simulink model "ASM_Traffic"  (R2026a)
settings: Solver=ode1  StartTime=SIM.tstart.v  StopTime=SIM.tend.v  FixedStep=SIM.StepSize.v
PostLoadFcn:
  | if any(exist('dsrtsu_mdlpostloadfcn', 'file') ~= 0), dsrtsu_mdlpostloadfcn('Execute', bdroot); end
  | try, asm_mdl_postloadfcn(bdroot, 'UpdateModel', 3600); catch, disp(lasterr); end,
InitFcn:
  | , if any(exist('rtifpga_mdlclblib', 'file') ~= 0), rtifpga_mdlclblib('Init', bdroot); end,
  | , if any(exist('dsmpb_private', 'file') ~= 0), dsmpb_private('dsmpb_mdlclblib', 'Init', bdroot); end,
model workspace (MAT data in the model file):
  asmReferencePath = [0 0.01 0.02 0.03 0.04 0.05 0.06 0.07 0.08 0.09 0.1 0.11 ... (350007 elements, 50001x7)]
  roadBounds : Simulink.Parameter (value not decoded)
  safetyAxes : Simulink.Parameter (value not decoded)
undefined symbols (not defined in the file): _to_, a0b2, ASM_BrakeHydraulics_DemoSystems, ASM_VehicleDynamics_DemoSystems, b98103fe8ad365046cd0, BrakeCircuit, controllerConfig, CPT, Crankshaft, DiscIntNeverNeededParam, dsmsi, FinalDriveAssembly, MDL, ModeSignals, mu, Pos_BrakePedal_Maneuver, rad, RefSignals, roadFamilyData, roadFamilyId, s_to_rpm, SIM, SoftECU, Suspension, Tire, Transmission
libraries: ASM_Traffic_lib x135, simulink x98, ASM_Utils_lib x77, ASM_VehicleDynamics_lib x70, ASM_Environment_lib x22, dsmpblib x20, dsmsilib x15, MDLD_Utils_lib x10, ASM_BrakeHydraulics_lib x3, sl_discontinuities x2
(part 40 of 65)

== system ASM_Traffic/Environment/Road/UserInterface/PAR_Plant/Pos_CP_CoorsSys_E[:][x;y][m] ==
  Pos_CP[x;y][m] : Inport
  Active_CP_VehDyn_Trailer[] : Inport  Port=2
  Bus Selector : BusSelector  OutputSignals=Pos_CP_FL_CoorSys_E[x;y][m],Pos_CP_FR_CoorSys_E[x;y][m],Pos_CP_RL_CoorSys_E[x;y][m],Pos_CP_RL2_CoorSys_E[x;y][m],Pos_CP_RR_CoorSys_E[x;y][m],Pos_CP_RR2_CoorSys_E[x;y][m],Pos_CP_R2L_CoorSys_E[x;y][m],Pos_CP_R2L2_CoorSys_E[x;y][m],Pos_CP_R2R_CoorSys_E[x;y][m],Pos_CP_R2R2_CoorSys_E[x;y][m],Pos_CP_FL_Trailer_CoorSys_E[x;y][m],Pos_CP_FL2_Trailer_CoorSys_E[x;y][m],Pos_CP_FR_Trailer_CoorSys_E[x;y][m],Pos_CP_FR2_Trailer_CoorSys_E[x;y][m],Pos_CP_RL_Trailer_CoorSys_E[x;y][m],Pos_CP_RL2_Trailer_CoorSys_E[x;y][m],Pos_CP_RR_Trailer_CoorSys_E[x;y][m],Pos_CP_RR2_Trailer_CoorSys_E[x;y][m],Pos_CP_R2L_Trailer_CoorSys_E[x;y][m],Pos_CP_R2L2_Trailer_CoorSys_E[x;y][m],Pos_CP_R2R_Trailer_CoorSys_E[x;y][m],Pos_CP_R2R2_Trailer_CoorSys_E[x;y][m],Pos_CP_Front_CoorSys_E[x;y][m],Pos_CP_Rear_CoorSys_E[x;y][m]
  Mux : Mux  Inputs=24
  Selector : Selector  IndexOptions=Index vector (port)  Indices=[1 3]  OutputSizes=1
  Pos_CP_CoorsSys_E[:][x;y][m] : Outport  VectorParamsAs1DForOutWhenUnconnected=off
  wires:
  Bus Selector/24 -> Mux/24  "<Pos_CP_Rear_CoorSys_E[x;y][m]>"
  Bus Selector/23 -> Mux/23  "<Pos_CP_Front_CoorSys_E[x;y][m]>"
  Selector/1 -> Pos_CP_CoorsSys_E[:][x;y][m]/1
  Active_CP_VehDyn_Trailer[]/1 -> Selector/2
  Pos_CP[x;y][m]/1 -> Bus Selector/1
  Bus Selector/1 -> Mux/1  "<Pos_CP_FL_CoorSys_E[x;y][m]>"
  Bus Selector/2 -> Mux/2  "<Pos_CP_FR_CoorSys_E[x;y][m]>"
  Bus Selector/3 -> Mux/3  "<Pos_CP_RL_CoorSys_E[x;y][m]>"
  Bus Selector/4 -> Mux/4  "<Pos_CP_RL2_CoorSys_E[x;y][m]>"
  Bus Selector/5 -> Mux/5  "<Pos_CP_RR_CoorSys_E[x;y][m]>"
  Bus Selector/6 -> Mux/6  "<Pos_CP_RR2_CoorSys_E[x;y][m]>"
  Bus Selector/7 -> Mux/7  "<Pos_CP_R2L_CoorSys_E[x;y][m]>"
  Bus Selector/8 -> Mux/8  "<Pos_CP_R2L2_CoorSys_E[x;y][m]>"
  Bus Selector/9 -> Mux/9  "<Pos_CP_R2R_CoorSys_E[x;y][m]>"
  Bus Selector/10 -> Mux/10  "<Pos_CP_R2R2_CoorSys_E[x;y][m]>"
  Bus Selector/11 -> Mux/11  "<Pos_CP_FL_Trailer_CoorSys_E[x;y][m]>"
  Bus Selector/12 -> Mux/12  "<Pos_CP_FL2_Trailer_CoorSys_E[x;y][m]>"
  Bus Selector/13 -> Mux/13  "<Pos_CP_FR_Trailer_CoorSys_E[x;y][m]>"
  Bus Selector/14 -> Mux/14  "<Pos_CP_FR2_Trailer_CoorSys_E[x;y][m]>"
  Bus Selector/15 -> Mux/15  "<Pos_CP_RL_Trailer_CoorSys_E[x;y][m]>"
  Bus Selector/16 -> Mux/16  "<Pos_CP_RL2_Trailer_CoorSys_E[x;y][m]>"
  Bus Selector/17 -> Mux/17  "<Pos_CP_RR_Trailer_CoorSys_E[x;y][m]>"
  Bus Selector/18 -> Mux/18  "<Pos_CP_RR2_Trailer_CoorSys_E[x;y][m]>"
  Bus Selector/19 -> Mux/19  "<Pos_CP_R2L_Trailer_CoorSys_E[x;y][m]>"
  Bus Selector/20 -> Mux/20  "<Pos_CP_R2L2_Trailer_CoorSys_E[x;y][m]>"
  Bus Selector/21 -> Mux/21  "<Pos_CP_R2R_Trailer_CoorSys_E[x;y][m]>"
  Bus Selector/22 -> Mux/22  "<Pos_CP_R2R2_Trailer_CoorSys_E[x;y][m]>"
  Mux/1 -> Selector/1

== system ASM_Traffic/Environment/Sensors/PlantModel/Collision_Sensor/ASMSignalCollector ==
  Bus Creator3 : BusCreator  Inputs=1
  tag scope: ASMBUS_Environment_Traffic_Sensors_Collision_Sensor=scoped
  wires:
  [ASMBUS_Traf_Sensors_Collision_Sensor_1] -> Bus Creator3/1  "Collision_Sensor_1"
  Bus Creator3/1 -> [ASMBUS_Environment_Traffic_Sensors_Collision_Sensor]  "Collision_Sensor"

== system ASM_Traffic/Environment/Sensors/PlantModel/Collision_Sensor/Enable_Collision_Sensor ==
  Enable_In[0Off|1On] : Inport
  Constant : Constant  Value=0.5  SampleTime=-1
  Constant1 : Constant  SampleTime=-1
  Constant2 : Constant  Value=0  SampleTime=-1
  Enable_Sensor : Gain
  Multiport Switch : MultiPortSwitch  DataPortOrder=Zero-based contiguous  Inputs=2  zeroidx=on  SaturateOnIntegerOverflow=off  InputSameDT=off
  Relational Operator : RelationalOperator  Operator=>  OutDataTypeStr=boolean  InputSameDT=off
  Enable_Out[0Off|1On] : Outport  VectorParamsAs1DForOutWhenUnconnected=off
  wires:
  Enable_In[0Off|1On]/1 -> Enable_Sensor/1
  Enable_Sensor/1 -> Relational Operator/1
  Relational Operator/1 -> Multiport Switch/1
  Multiport Switch/1 -> Enable_Out[0Off|1On]/1
  Constant/1 -> Relational Operator/2
  Constant1/1 -> Multiport Switch/3
  Constant2/1 -> Multiport Switch/2

== system ASM_Traffic/Environment/Sensors/PlantModel/Collision_Sensor/ExternalUserData ==
  Flag_CollsionSensor_Parameters_Used[0|1] : Constant  Value=[0]
  Pos_x_CollisionObj_Custom_RefPnt[m] : Constant  Value=[0]
  Pos_y_CollisionObj_Custom_RefPnt[m] : Constant  Value=[0]
  TrafficObject_Type_CollisionObj[] : Constant  Value=[0]
  Flag_CollsionSensor_Parameters_Used_External[0|1] : Outport  VectorParamsAs1DForOutWhenUnconnected=off
  TrafficObject_Type_CollisionObj_External[] : Outport  Port=2  VectorParamsAs1DForOutWhenUnconnected=off
  Pos_x_CollisionObj_Custom_RefPnt_External[m] : Outport  Port=3  VectorParamsAs1DForOutWhenUnconnected=off
  Pos_y_CollisionObj_Custom_RefPnt_External[m] : Outport  Port=4  VectorParamsAs1DForOutWhenUnconnected=off
  wires:
  TrafficObject_Type_CollisionObj[]/1 -> TrafficObject_Type_CollisionObj_External[]/1  "TrafficObject_Type_CollisionObj_External[]"
  Pos_y_CollisionObj_Custom_RefPnt[m]/1 -> Pos_y_CollisionObj_Custom_RefPnt_External[m]/1  "Pos_y_CollisionObj_Custom_RefPnt_External[m]"
  Flag_CollsionSensor_Parameters_Used[0|1]/1 -> Flag_CollsionSensor_Parameters_Used_External[0|1]/1  "Flag_CollsionSensor_Parameters_Used_External[0|1]"
  Pos_x_CollisionObj_Custom_RefPnt[m]/1 -> Pos_x_CollisionObj_Custom_RefPnt_External[m]/1  "Pos_x_CollisionObj_Custom_RefPnt_External[m]"

== system ASM_Traffic/Environment/Sensors/PlantModel/Collision_Sensor/GetFellowPositionVector ==
  <FellowPositions> : Inport
  Bus Selector11 : BusSelector  OutputSignals=Pos_Fellows_MainPnt_CoorSys_E[x;y;z][m].Pos_x_Fellows[m],Pos_Fellows_MainPnt_CoorSys_E[x;y;z][m].Pos_y_Fellows[m],Pos_Fellows_MainPnt_CoorSys_E[x;y;z][m].Pos_z_Fellows[m],Angle_Fellows[x;y;z][deg].Angle_Roll_Fellows[deg],Angle_Fellows[x;y;z][deg].Angle_Pitch_Fellows[deg],Angle_Fellows[x;y;z][deg].Angle_Yaw_Fellows[deg]
  Mux1 : Mux  Inputs=3
  Mux2 : Mux  Inputs=3
  Pos_Fellows_MainPnt_CoorSys_E[x;y;z][m] : Outport  VectorParamsAs1DForOutWhenUnconnected=off
  Angle_Fellows[deg] : Outport  Port=2  VectorParamsAs1DForOutWhenUnconnected=off
  wires:
  Mux2/1 -> Pos_Fellows_MainPnt_CoorSys_E[x;y;z][m]/1  "Pos_Fellows_MainPnt_CoorSys_E[x;y;z][m]"
  Mux1/1 -> Angle_Fellows[deg]/1  "Pos_Fellows_MainPnt_CoorSys_E_vec"
  Bus Selector11/4 -> Mux1/1  "<Angle_Roll_Fellows[deg]>"
  Bus Selector11/1 -> Mux2/1  "<Pos_x_Fellows[m]>"
  Bus Selector11/2 -> Mux2/2  "<Pos_y_Fellows[m]>"
  Bus Selector11/6 -> Mux1/3  "<Angle_Yaw_Fellows[deg]>"
  Bus Selector11/5 -> Mux1/2  "<Angle_Pitch_Fellows[deg]>"
  <FellowPositions>/1 -> Bus Selector11/1
  Bus Selector11/3 -> Mux2/3  "<Pos_z_Fellows[m]>"

== system ASM_Traffic/Environment/Sensors/PlantModel/Line_Sensor/ASMSignalCollector ==
  note: LineSensor-Output not
      | fed into SignalBus due
      | to large amount of signal data.
  Add{,1..5} (6 alike) : Sum
  Bus Creator1 : BusCreator  Inputs=8
  Bus Creator{2,4..8} (6 alike) : BusCreator  Inputs=3
  Bus Creator3 : BusCreator  Inputs=1
  Bus Selector : BusSelector  OutputSignals=SensorOutput.Info,SensorOutput.Road,SensorOutput.Junction
  Bus Selector1 : BusSelector  OutputSignals=Road_Lanes.Pos_x_Road_Lanes_CoorSys_E[m],Road_Lanes.Pos_y_Road_Lanes_CoorSys_E[m],Road_Lanes.Pos_z_Road_Lanes_CoorSys_E[m]
  Bus Selector2 : BusSelector  OutputSignals=Junction_Borders.Pos_x_Junction_Borders_CoorSys_E[m],Junction_Borders.Pos_y_Junction_Borders_CoorSys_E[m],Junction_Borders.Pos_z_Junction_Borders_CoorSys_E[m]
  Bus Selector3 : BusSelector  OutputSignals=Road_Shape_Lines.Pos_x_Road_Shape_Lines_CoorSys_E[m],Road_Shape_Lines.Pos_y_Road_Shape_Lines_CoorSys_E[m],Road_Shape_Lines.Pos_z_Road_Shape_Lines_CoorSys_E[m]
  Bus Selector4 : BusSelector  OutputSignals=Road_Shape_ContObj.Pos_x_Road_Shape_ContObj_CoorSys_E[m],Road_Shape_ContObj.Pos_y_Road_Shape_ContObj_CoorSys_E[m],Road_Shape_ContObj.Pos_z_Road_Shape_ContObj_CoorSys_E[m]
  Bus Selector5 : BusSelector  OutputSignals=Junction_Shape_Lines.Pos_x_Junction_Shape_Lines_CoorSys_E[m],Junction_Shape_Lines.Pos_y_Junction_Shape_Lines_CoorSys_E[m],Junction_Shape_Lines.Pos_z_Junction_Shape_Lines_CoorSys_E[m]
  Bus Selector6 : BusSelector  OutputSignals=Junction_Shape_ContObj.Pos_x_Junction_Shape_ContObj_CoorSys_E[m],Junction_Shape_ContObj.Pos_y_Junction_Shape_ContObj_CoorSys_E[m],Junction_Shape_ContObj.Pos_z_Junction_Shape_ContObj_CoorSys_E[m]
  Dummy : Constant  Value=0
  Idx_Vector_Junction_Borders : Constant  Value=1:1:60
  Idx_Vector_Junction_Shape_ContObj : Constant  Value=1:1:60
  Idx_Vector_Junction_Shape_Lines : Constant  Value=1:1:60
  Idx_Vector_Road_Lanes : Constant  Value=1:1:60
  Idx_Vector_Road_Shape_ContObj : Constant  Value=1:1:60
  Idx_Vector_Road_Shape_Lines : Constant  Value=1:1:60
  Saturation : Saturate  UpperLimit=MDL.Traffic.Sensors.LineSensor.Const_Road_Lane_Output_Dimension.v  LowerLimit=1
  Saturation1 : Saturate  UpperLimit=MDL.Traffic.Sensors.LineSensor.Const_Road_Shape_Line_Output_Dimension.v  LowerLimit=1
  Saturation2 : Saturate  UpperLimit=MDL.Traffic.Sensors.LineSensor.Const_Road_Shape_ContObj_Output_Dimension.v  LowerLimit=1
  Saturation3 : Saturate  UpperLimit=MDL.Traffic.Sensors.LineSensor.Const_Junction_Border_Output_Dimension.v  LowerLimit=1
  Saturation4 : Saturate  UpperLimit=MDL.Traffic.Sensors.LineSensor.Const_Junction_Border_Output_Dimension.v  LowerLimit=1
  Saturation5 : Saturate  UpperLimit=MDL.Traffic.Sensors.LineSensor.Const_Junction_Border_Output_Dimension.v  LowerLimit=1
  Selector1 : Selector  InputPortWidth=MDL.Traffic.Sensors.LineSensor.Const_Road_Lane_Output_Dimension.v  IndexOptions=Index vector (port)  Indices=1  OutputSizes=36
  Selector10 : Selector  InputPortWidth=MDL.Traffic.Sensors.LineSensor.Const_Road_Shape_ContObj_Output_Dimension.v  IndexOptions=Index vector (port)  Indices=1  OutputSizes=36
  Selector11 : Selector  InputPortWidth=MDL.Traffic.Sensors.LineSensor.Const_Road_Shape_ContObj_Output_Dimension.v  IndexOptions=Index vector (port)  Indices=1  OutputSizes=36
  Selector12 : Selector  InputPortWidth=MDL.Traffic.Sensors.LineSensor.Const_Road_Shape_ContObj_Output_Dimension.v  IndexOptions=Index vector (port)  Indices=1  OutputSizes=36
  Selector13 : Selector  InputPortWidth=MDL.Traffic.Sensors.LineSensor.Const_Junction_Shape_Line_Output_Dimension.v  IndexOptions=Index vector (port)  Indices=1  OutputSizes=36
  Selector14 : Selector  InputPortWidth=MDL.Traffic.Sensors.LineSensor.Const_Junction_Shape_Line_Output_Dimension.v  IndexOptions=Index vector (port)  Indices=1  OutputSizes=36
  Selector15 : Selector  InputPortWidth=MDL.Traffic.Sensors.LineSensor.Const_Junction_Shape_Line_Output_Dimension.v  IndexOptions=Index vector (port)  Indices=1  OutputSizes=36
  Selector16 : Selector  InputPortWidth=MDL.Traffic.Sensors.LineSensor.Const_Junction_Shape_ContObj_Output_Dimension.v  IndexOptions=Index vector (port)  Indices=1  OutputSizes=36
  Selector17 : Selector  InputPortWidth=MDL.Traffic.Sensors.LineSensor.Const_Junction_Shape_ContObj_Output_Dimension.v  IndexOptions=Index vector (port)  Indices=1  OutputSizes=36
  Selector18 : Selector  InputPortWidth=MDL.Traffic.Sensors.LineSensor.Const_Junction_Shape_ContObj_Output_Dimension.v  IndexOptions=Index vector (port)  Indices=1  OutputSizes=36
  Selector2 : Selector  InputPortWidth=MDL.Traffic.Sensors.LineSensor.Const_Road_Lane_Output_Dimension.v  IndexOptions=Index vector (port)  Indices=1  OutputSizes=36
  Selector3 : Selector  InputPortWidth=MDL.Traffic.Sensors.LineSensor.Const_Road_Lane_Output_Dimension.v  IndexOptions=Index vector (port)  Indices=1  OutputSizes=36
  Selector4 : Selector  InputPortWidth=MDL.Traffic.Sensors.LineSensor.Const_Junction_Border_Output_Dimension.v  IndexOptions=Index vector (port)  Indices=1  OutputSizes=36
  Selector5 : Selector  InputPortWidth=MDL.Traffic.Sensors.LineSensor.Const_Junction_Border_Output_Dimension.v  IndexOptions=Index vector (port)  Indices=1  OutputSizes=36
  Selector6 : Selector  InputPortWidth=MDL.Traffic.Sensors.LineSensor.Const_Junction_Border_Output_Dimension.v  IndexOptions=Index vector (port)  Indices=1  OutputSizes=36
  Selector7 : Selector  InputPortWidth=MDL.Traffic.Sensors.LineSensor.Const_Road_Shape_Line_Output_Dimension.v  IndexOptions=Index vector (port)  Indices=1  OutputSizes=36
  Selector8 : Selector  InputPortWidth=MDL.Traffic.Sensors.LineSensor.Const_Road_Shape_Line_Output_Dimension.v  IndexOptions=Index vector (port)  Indices=1  OutputSizes=36
  Selector9 : Selector  InputPortWidth=MDL.Traffic.Sensors.LineSensor.Const_Road_Shape_Line_Output_Dimension.v  IndexOptions=Index vector (port)  Indices=1  OutputSizes=36
  Signal Specification{,1..5} (6 alike) : SignalSpecification  Dimensions=60
  z_Offset[m] : Constant  Value=0.1
  tag scope: ASMBUS_Environment_Traffic_Sensors_Line_Sensor=scoped
  wires:
  Dummy/1 -> Bus Creator1/8  "Dummy_SensorOutput"
  Saturation5/1 -> Signal Specification5/1
  Idx_Vector_Junction_Shape_ContObj/1 -> Saturation5/1
  Signal Specification5/1 -> Selector18/2, Selector16/2, Selector17/2
  Bus Creator8/1 -> Bus Creator1/7  "Pos_Junction_Shape_ContObj_Animation_CoorSys_E"
  Add4/1 -> Bus Creator8/3  "Pos_z_Junction_Shape_ContObj_Animation_CoorSys_E"
  Selector17/1 -> Add4/1
  Selector16/1 -> Bus Creator8/2  "Pos_y_Junction_Shape_ContObj_Animation_CoorSys_E"
  Selector18/1 -> Bus Creator8/1  "Pos_x_Junction_Shape_ContObj_Animation_CoorSys_E"
  Bus Selector6/3 -> Selector17/1  "<Pos_z_Junction_Shape_ContObj_CoorSys_E[m]>"
  Bus Selector6/2 -> Selector16/1  "<Pos_y_Junction_Shape_ContObj_CoorSys_E[m]>"
  Bus Selector6/1 -> Selector18/1  "<Pos_x_Junction_Shape_ContObj_CoorSys_E[m]>"
  Bus Selector/3 -> Bus Selector2/1, Bus Selector5/1, Bus Selector6/1  "<Junction>"
  Saturation4/1 -> Signal Specification4/1
  Idx_Vector_Junction_Shape_Lines/1 -> Saturation4/1
  Signal Specification4/1 -> Selector15/2, Selector13/2, Selector14/2
  Bus Creator7/1 -> Bus Creator1/6  "Pos_Junction_Shape_Line_Animation_CoorSys_E"
  Add5/1 -> Bus Creator7/3  "Pos_z_Junction_Shape_Line_Animation_CoorSys_E"
  Selector14/1 -> Add5/1
  Selector13/1 -> Bus Creator7/2  "Pos_y_Junction_Shape_Line_Animation_CoorSys_E"
  Selector15/1 -> Bus Creator7/1  "Pos_x_Junction_Shape_Line_Animation_CoorSys_E"
  Bus Selector5/3 -> Selector14/1  "<Pos_z_Junction_Shape_Lines_CoorSys_E[m]>"
  Bus Selector5/2 -> Selector13/1  "<Pos_y_Junction_Shape_Lines_CoorSys_E[m]>"
  Bus Selector5/1 -> Selector15/1  "<Pos_x_Junction_Shape_Lines_CoorSys_E[m]>"
  Signal Specification3/1 -> Selector6/2, Selector4/2, Selector5/2
  Saturation3/1 -> Signal Specification3/1
  Idx_Vector_Junction_Borders/1 -> Saturation3/1
  Signal Specification2/1 -> Selector12/2, Selector10/2, Selector11/2
  Saturation2/1 -> Signal Specification2/1
  Idx_Vector_Road_Shape_ContObj/1 -> Saturation2/1
  Signal Specification1/1 -> Selector9/2, Selector7/2, Selector8/2
  Saturation1/1 -> Signal Specification1/1
  Idx_Vector_Road_Shape_Lines/1 -> Saturation1/1
  Signal Specification/1 -> Selector2/2, Selector1/2, Selector3/2
  Bus Creator4/1 -> Bus Creator1/5  "Pos_Junction_Border_Animation_CoorSys_E"
  Bus Creator6/1 -> Bus Creator1/4  "Pos_Road_Shape_ContObj_Animation_CoorSys_E"
  Bus Creator5/1 -> Bus Creator1/3  "Pos_Road_Shape_Line_Animation_CoorSys_E"
  Add2/1 -> Bus Creator6/3  "Pos_z_Road_Shape_ContObj_Animation_CoorSys_E"
  Selector11/1 -> Add2/1
  Selector10/1 -> Bus Creator6/2  "Pos_y_Road_Shape_ContObj_Animation_CoorSys_E"
  Selector12/1 -> Bus Creator6/1  "Pos_x_Road_Shape_ContObj_Animation_CoorSys_E"
  Bus Selector4/3 -> Selector11/1  "<Pos_z_Road_Shape_ContObj_CoorSys_E[m]>"
  Bus Selector4/2 -> Selector10/1  "<Pos_y_Road_Shape_ContObj_CoorSys_E[m]>"
  Bus Selector4/1 -> Selector12/1  "<Pos_x_Road_Shape_ContObj_CoorSys_E[m]>"
  Bus Selector/2 -> Bus Selector1/1, Bus Selector3/1, Bus Selector4/1  "<Road>"
  z_Offset[m]/1 -> Add4/2, Add3/2, Add/2, Add2/2, Add1/2, Add5/2
  Add3/1 -> Bus Creator5/3  "Pos_z_Road_Shape_Line_Animation_CoorSys_E"
  Selector8/1 -> Add3/1
  Selector7/1 -> Bus Creator5/2  "Pos_y_Road_Shape_Line_Animation_CoorSys_E"
  Selector9/1 -> Bus Creator5/1  "Pos_x_Road_Shape_Line_Animation_CoorSys_E"
  Bus Selector3/3 -> Selector8/1  "<Pos_z_Road_Shape_Lines_CoorSys_E[m]>"
  Bus Selector3/2 -> Selector7/1  "<Pos_y_Road_Shape_Lines_CoorSys_E[m]>"
  Bus Selector3/1 -> Selector9/1  "<Pos_x_Road_Shape_Lines_CoorSys_E[m]>"
  Add1/1 -> Bus Creator4/3  "Pos_z_Junction_Border_Animation_CoorSys_E"
  Selector5/1 -> Add1/1
  Selector4/1 -> Bus Creator4/2  "Pos_y_Junction_Border_Animation_CoorSys_E"
  Selector6/1 -> Bus Creator4/1  "Pos_x_Junction_Border_Animation_CoorSys_E"
  Bus Selector2/3 -> Selector5/1  "<Pos_z_Junction_Borders_CoorSys_E[m]>"
  Bus Selector2/2 -> Selector4/1  "<Pos_y_Junction_Borders_CoorSys_E[m]>"
  Bus Selector2/1 -> Selector6/1  "<Pos_x_Junction_Borders_CoorSys_E[m]>"
  Saturation/1 -> Signal Specification/1
  Add/1 -> Bus Creator2/3  "Pos_z_Road_Lane_Animation_CoorSys_E"
  Idx_Vector_Road_Lanes/1 -> Saturation/1
  Bus Creator2/1 -> Bus Creator1/2  "Pos_Road_Lane_Animation_CoorSys_E"
  Selector2/1 -> Add/1
  Selector1/1 -> Bus Creator2/2  "Pos_y_Road_Lane_Animation_CoorSys_E"
  Selector3/1 -> Bus Creator2/1  "Pos_x_Road_Lane_Animation_CoorSys_E"
  Bus Selector1/3 -> Selector2/1  "<Pos_z_Road_Lanes_CoorSys_E[m]>"
  Bus Selector1/2 -> Selector1/1  "<Pos_y_Road_Lanes_CoorSys_E[m]>"
  Bus Selector1/1 -> Selector3/1  "<Pos_x_Road_Lanes_CoorSys_E[m]>"
  Bus Creator1/1 -> Bus Creator3/1  "Line_Sensor_1"
  Bus Selector/1 -> Bus Creator1/1  "<Info>"
  Bus Creator3/1 -> [ASMBUS_Environment_Traffic_Sensors_Line_Sensor]  "Line_Sensor"
  [ASMBUS_Traf_Sensors_Line_Sensor_1] -> Bus Selector/1

== system ASM_Traffic/Environment/Sensors/PlantModel/Line_Sensor/Enable_Line_Sensor ==
  Enable_In[0Off|1On] : Inport
  Constant : Constant  Value=0.5  SampleTime=-1
  Constant1 : Constant  SampleTime=-1
  Constant2 : Constant  Value=0  SampleTime=-1
  Enable_Sensor : Gain
  Multiport Switch : MultiPortSwitch  DataPortOrder=Zero-based contiguous  Inputs=2  zeroidx=on  SaturateOnIntegerOverflow=off  InputSameDT=off
  Relational Operator : RelationalOperator  Operator=>  OutDataTypeStr=boolean  InputSameDT=off
  Enable_Out[0Off|1On] : Outport  VectorParamsAs1DForOutWhenUnconnected=off
  wires:
  Constant2/1 -> Multiport Switch/2
  Constant1/1 -> Multiport Switch/3
  Constant/1 -> Relational Operator/2
  Multiport Switch/1 -> Enable_Out[0Off|1On]/1
  Relational Operator/1 -> Multiport Switch/1
  Enable_Sensor/1 -> Relational Operator/1
  Enable_In[0Off|1On]/1 -> Enable_Sensor/1

== system ASM_Traffic/Environment/Sensors/PlantModel/Object_Sensor_2D/ASMSignalCollector ==
  Bus Creator1 : BusCreator  Inputs=10
  Bus Creator{2..4,6..9} (7 alike) : BusCreator  Inputs=6
  Bus Selector{,1,3..7} (7 alike) : BusSelector  OutputSignals=SensorIndex,SensorStatus,SensorOutput
  Bus Selector10 : BusSelector  OutputSignals=Sensor2
  Bus Selector11 : BusSelector  OutputSignals=Sensor2
  Bus Selector12 : BusSelector  OutputSignals=Sensor2
  Bus Selector13 : BusSelector  OutputSignals=Sensor3
  Bus Selector14 : BusSelector  OutputSignals=Sensor3
  Bus Selector15 : BusSelector  OutputSignals=Sensor3
  Bus Selector16 : BusSelector  OutputSignals=Sensor4
  Bus Selector17 : BusSelector  OutputSignals=Sensor4
  Bus Selector18 : BusSelector  OutputSignals=Sensor4
  Bus Selector19 : BusSelector  OutputSignals=Sensor5
  Bus Selector2 : BusSelector  OutputSignals=Sensor1
  Bus Selector20 : BusSelector  OutputSignals=Sensor5
  Bus Selector21 : BusSelector  OutputSignals=Sensor5
  Bus Selector22 : BusSelector  OutputSignals=Sensor6
  Bus Selector23 : BusSelector  OutputSignals=Sensor6
  Bus Selector24 : BusSelector  OutputSignals=Sensor6
  Bus Selector25 : BusSelector  OutputSignals=Sensor7
  Bus Selector26 : BusSelector  OutputSignals=Sensor7
  Bus Selector27 : BusSelector  OutputSignals=Sensor7
  Bus Selector28 : BusSelector  OutputSignals=Sensors_2D_Common
  Bus Selector8 : BusSelector  OutputSignals=Sensor1
  Bus Selector9 : BusSelector  OutputSignals=Sensor1
  Rename : Subsystem
  Rename1 : Subsystem
  Rename10 : Subsystem
  Rename11 : Subsystem
  Rename12 : Subsystem
  Rename13 : Subsystem
  Rename2 : Subsystem
  Rename3 : Subsystem
  Rename4 : Subsystem
  Rename5 : Subsystem
  Rename6 : Subsystem
  Rename7 : Subsystem
  Rename8 : Subsystem
  Rename9 : Subsystem
  tag scope: ASMBUS_Environment_Traffic_Sensors_Object_Sensor_2D=scoped
  wires:
  Rename13/1(Out1) -> Bus Creator9/6  "ObjectData"
  Rename12/1(Out1) -> Bus Creator4/6  "ObjectData"
  Rename11/1(Out1) -> Bus Creator8/6  "ObjectData"
  Rename10/1(Out1) -> Bus Creator7/6  "ObjectData"
  Rename9/1(Out1) -> Bus Creator6/6  "ObjectData"
  Rename8/1(Out1) -> Bus Creator3/6  "ObjectData"
  Rename7/1(Out1) -> Bus Creator9/1  "Parameters"
  Rename6/1(Out1) -> Bus Creator4/1  "Parameters"
  Rename5/1(Out1) -> Bus Creator8/1  "Parameters"
  Rename4/1(Out1) -> Bus Creator7/1  "Parameters"
  Rename3/1(Out1) -> Bus Creator6/1  "Parameters"
  Rename2/1(Out1) -> Bus Creator3/1  "Parameters"
  Rename1/1(Out1) -> Bus Creator2/6  "ObjectData"
  Rename/1(Out1) -> Bus Creator2/1  "Parameters"
  [ASMBUS_Environment_Traffic_2DObjSensor_ObjectData] -> Bus Selector27/1
  [ASMBUS_Environment_Traffic_2DObjSensor_SensorSignals] -> Bus Selector26/1
  [ASMBUS_Environment_Traffic_2DObjSensor_Parameter] -> Bus Selector25/1
  [ASMBUS_Environment_Traffic_2DObjSensor_ObjectData] -> Bus Selector24/1
  [ASMBUS_Environment_Traffic_2DObjSensor_SensorSignals] -> Bus Selector23/1
  [ASMBUS_Environment_Traffic_2DObjSensor_Parameter] -> Bus Selector22/1
  [ASMBUS_Environment_Traffic_2DObjSensor_ObjectData] -> Bus Selector21/1
  [ASMBUS_Environment_Traffic_2DObjSensor_SensorSignals] -> Bus Selector20/1
  [ASMBUS_Environment_Traffic_2DObjSensor_Parameter] -> Bus Selector19/1
  [ASMBUS_Environment_Traffic_2DObjSensor_ObjectData] -> Bus Selector18/1
  [ASMBUS_Environment_Traffic_2DObjSensor_SensorSignals] -> Bus Selector17/1
  [ASMBUS_Environment_Traffic_2DObjSensor_Parameter] -> Bus Selector16/1
  [ASMBUS_Environment_Traffic_2DObjSensor_ObjectData] -> Bus Selector15/1
  [ASMBUS_Environment_Traffic_2DObjSensor_SensorSignals] -> Bus Selector14/1
  [ASMBUS_Environment_Traffic_2DObjSensor_Parameter] -> Bus Selector13/1
  [ASMBUS_Environment_Traffic_2DObjSensor_ObjectData] -> Bus Selector12/1
  [ASMBUS_Environment_Traffic_2DObjSensor_SensorSignals] -> Bus Selector11/1
  [ASMBUS_Environment_Traffic_2DObjSensor_Parameter] -> Bus Selector10/1
  Bus Selector9/1 -> Rename1/1(In1)  "<Sensor1>"
  Bus Selector8/1 -> Bus Selector/1  "<Sensor1>"
  Bus Selector2/1 -> Rename/1(In1)  "<Sensor1>"
  Bus Selector27/1 -> Rename13/1(In1)  "<Sensor7>"
  Bus Selector24/1 -> Rename12/1(In1)  "<Sensor6>"
  Bus Selector21/1 -> Rename11/1(In1)  "<Sensor5>"
  Bus Selector18/1 -> Rename10/1(In1)  "<Sensor4>"
  Bus Selector15/1 -> Rename9/1(In1)  "<Sensor3>"
  Bus Selector12/1 -> Rename8/1(In1)  "<Sensor2>"
  [ASMBUS_Environment_Traffic_2DObjSensor_ObjectData] -> Bus Selector9/1
  Bus Selector1/3 -> Bus Creator4/4  "<SensorOutput>"
  Bus Selector1/2 -> Bus Creator4/3  "<SensorStatus>"
  Bus Selector1/1 -> Bus Creator4/2  "<SensorIndex>"
  Bus Selector22/1 -> Rename6/1(In1)  "<Sensor6>"
  Bus Creator4/1 -> Bus Creator1/9  "Sensor_6_Right"
  Bus Selector23/1 -> Bus Selector1/1  "<Sensor6>"
  Bus Selector7/3 -> Bus Creator9/4  "<SensorOutput>"
  Bus Selector7/2 -> Bus Creator9/3  "<SensorStatus>"
  Bus Selector7/1 -> Bus Creator9/2  "<SensorIndex>"
  Bus Selector25/1 -> Rename7/1(In1)  "<Sensor7>"
  Bus Creator9/1 -> Bus Creator1/10  "Sensor_7_Rear_Right"
  Bus Selector26/1 -> Bus Selector7/1  "<Sensor7>"
  Bus Selector6/3 -> Bus Creator8/4  "<SensorOutput>"
  Bus Selector6/2 -> Bus Creator8/3  "<SensorStatus>"
  Bus Selector6/1 -> Bus Creator8/2  "<SensorIndex>"
  Bus Selector19/1 -> Rename5/1(In1)  "<Sensor5>"
  Bus Creator8/1 -> Bus Creator1/8  "Sensor_5_Front_Right"
  Bus Selector20/1 -> Bus Selector6/1  "<Sensor5>"
  Bus Selector5/3 -> Bus Creator7/4  "<SensorOutput>"
  Bus Selector5/2 -> Bus Creator7/3  "<SensorStatus>"
  Bus Selector5/1 -> Bus Creator7/2  "<SensorIndex>"
  Bus Selector16/1 -> Rename4/1(In1)  "<Sensor4>"
  Bus Creator7/1 -> Bus Creator1/7  "Sensor_4_Rear_Left"
  Bus Selector17/1 -> Bus Selector5/1  "<Sensor4>"
  Bus Selector4/3 -> Bus Creator6/4  "<SensorOutput>"
  Bus Selector4/2 -> Bus Creator6/3  "<SensorStatus>"
  Bus Selector4/1 -> Bus Creator6/2  "<SensorIndex>"
  Bus Selector13/1 -> Rename3/1(In1)  "<Sensor3>"
  Bus Creator6/1 -> Bus Creator1/6  "Sensor_3_Left"
  Bus Selector14/1 -> Bus Selector4/1  "<Sensor3>"
  Bus Selector3/3 -> Bus Creator3/4  "<SensorOutput>"
  Bus Selector3/2 -> Bus Creator3/3  "<SensorStatus>"
  Bus Selector3/1 -> Bus Creator3/2  "<SensorIndex>"
  Bus Selector10/1 -> Rename2/1(In1)  "<Sensor2>"
  Bus Creator3/1 -> Bus Creator1/5  "Sensor_2_Front_Left"
  Bus Selector11/1 -> Bus Selector3/1  "<Sensor2>"
  Bus Selector/3 -> Bus Creator2/4  "<SensorOutput>"
  Bus Selector/2 -> Bus Creator2/3  "<SensorStatus>"
  Bus Selector/1 -> Bus Creator2/2  "<SensorIndex>"
  [ASMBUS_Environment_Traffic_2DObjSensorCalc_Info] -> Bus Creator2/5, Bus Creator3/5, Bus Creator6/5, Bus Creator7/5, Bus Creator8/5, Bus Creator4/5, Bus Creator9/5  "Info"
  [ASMBUS_Environment_Traffic_SamplePulse_ObjectSensor2D] -> Bus Creator1/2  "Sample_Pulse"
  [ASMBUS_Environment_Traffic_SensorScheduler_ObjectSensor2D] -> Bus Creator1/3  "Sensor_Scheduler"
  [ASMBUS_Environment_Traffic_2DObjSensor_Parameter] -> Bus Selector2/1
  Bus Creator2/1 -> Bus Creator1/4  "Sensor_1_Front"
  [ASMBUS_Environment_Traffic_2DObjSensor_SensorSignals] -> Bus Selector8/1
  Bus Creator1/1 -> [ASMBUS_Environment_Traffic_Sensors_Object_Sensor_2D]  "Object_Sensor_2D"
  [ASMBUS_Environment_Traffic_2DObjSensor_Parameter] -> Bus Selector28/1
  Bus Selector28/1 -> Bus Creator1/1  "<Sensors_2D_Common>"

== system ASM_Traffic/Environment/Sensors/PlantModel/Object_Sensor_2D/Enable_Object_Sensor_2D ==
  Enable_In[0Off|1On] : Inport
  Constant : Constant  Value=0.5  SampleTime=-1
  Constant1 : Constant  SampleTime=-1
  Constant2 : Constant  Value=0  SampleTime=-1
  Enable_Sensor : Gain
  Multiport Switch : MultiPortSwitch  DataPortOrder=Zero-based contiguous  Inputs=2  zeroidx=on  SaturateOnIntegerOverflow=off  InputSameDT=off
  Relational Operator : RelationalOperator  Operator=>  OutDataTypeStr=boolean  InputSameDT=off
  Enable_Out[0Off|1On] : Outport  VectorParamsAs1DForOutWhenUnconnected=off
  wires:
  Constant2/1 -> Multiport Switch/2
  Constant1/1 -> Multiport Switch/3
  Constant/1 -> Relational Operator/2
  Multiport Switch/1 -> Enable_Out[0Off|1On]/1
  Relational Operator/1 -> Multiport Switch/1
  Enable_Sensor/1 -> Relational Operator/1
  Enable_In[0Off|1On]/1 -> Enable_Sensor/1

== system ASM_Traffic/Environment/Sensors/PlantModel/Object_Sensor_2D/ObjectData ==
  Traffic_Signals : Inport
  Road_Signals : Inport  Port=2
  Bus Creator : BusCreator  Inputs=7
  Bus Selector{1..3,5..8} (7 alike) : BusSelector  OutputSignals=SensorOutput.Object_ID[],SensorOutput.Object_Type[]
  Bus Selector4 : BusSelector  OutputSignals=Sensor_1_Front,Sensor_2_Front_Left,Sensor_3_Left,Sensor_4_Rear_Left,Sensor_5_Front_Right,Sensor_6_Right,Sensor_7_Rear_Right
  Sensor1 : Subsystem
  Sensor2 : Subsystem
  Sensor3 : Subsystem
  Sensor4 : Subsystem
  Sensor5 : Subsystem
  Sensor6 : Subsystem
  Sensor7 : Subsystem
  Terminator{1..21} (21 alike) : Terminator
  avoid_incomplete_trace2source : Subsystem
  avoid_incomplete_trace2source1 : Subsystem
  avoid_incomplete_trace2source10 : Subsystem
  avoid_incomplete_trace2source11 : Subsystem
  avoid_incomplete_trace2source12 : Subsystem
  avoid_incomplete_trace2source13 : Subsystem
  avoid_incomplete_trace2source2 : Subsystem
  avoid_incomplete_trace2source3 : Subsystem
  avoid_incomplete_trace2source4 : Subsystem
  avoid_incomplete_trace2source5 : Subsystem
  avoid_incomplete_trace2source6 : Subsystem
  avoid_incomplete_trace2source7 : Subsystem
  avoid_incomplete_trace2source8 : Subsystem
  avoid_incomplete_trace2source9 : Subsystem
  tag scope: ASMBUS_Environment_Traffic_2DObjSensor_ObjectData=scoped
  wires:
  avoid_incomplete_trace2source12/1(Out1) -> Sensor7/1(Object_ID[])
  avoid_incomplete_trace2source13/1(Out1) -> Sensor7/2(Object_Type[])
  avoid_incomplete_trace2source10/1(Out1) -> Sensor6/1(Object_ID[])
  avoid_incomplete_trace2source11/1(Out1) -> Sensor6/2(Object_Type[])
  avoid_incomplete_trace2source9/1(Out1) -> Sensor5/2(Object_Type[])
  avoid_incomplete_trace2source8/1(Out1) -> Sensor5/1(Object_ID[])
  avoid_incomplete_trace2source7/1(Out1) -> Sensor4/2(Object_Type[])
  avoid_incomplete_trace2source6/1(Out1) -> Sensor4/1(Object_ID[])
  avoid_incomplete_trace2source4/1(Out1) -> Sensor3/1(Object_ID[])
  avoid_incomplete_trace2source5/1(Out1) -> Sensor3/2(Object_Type[])
  avoid_incomplete_trace2source2/1(Out1) -> Sensor2/1(Object_ID[])
  avoid_incomplete_trace2source3/1(Out1) -> Sensor2/2(Object_Type[])
  avoid_incomplete_trace2source1/1(Out1) -> Sensor1/2(Object_Type[])
  avoid_incomplete_trace2source/1(Out1) -> Sensor1/1(Object_ID[])
  Bus Creator/1 -> [ASMBUS_Environment_Traffic_2DObjSensor_ObjectData]
  Sensor7/1(ASMSignalBus) -> Bus Creator/7  "Sensor7"
  Sensor6/1(ASMSignalBus) -> Bus Creator/6  "Sensor6"
  Sensor5/1(ASMSignalBus) -> Bus Creator/5  "Sensor5"
  Sensor4/1(ASMSignalBus) -> Bus Creator/4  "Sensor4"
  Sensor3/1(ASMSignalBus) -> Bus Creator/3  "Sensor3"
  Sensor2/1(ASMSignalBus) -> Bus Creator/2  "Sensor2"
  Sensor1/1(ASMSignalBus) -> Bus Creator/1  "Sensor1"
  Bus Selector4/7 -> Bus Selector8/1  "<Sensor_7_Rear_Right>"
  Bus Selector4/6 -> Bus Selector7/1  "<Sensor_6_Right>"
  Bus Selector4/5 -> Bus Selector6/1  "<Sensor_5_Front_Right>"
  Bus Selector4/4 -> Bus Selector5/1  "<Sensor_4_Rear_Left>"
  Bus Selector8/1 -> avoid_incomplete_trace2source12/1(In1)  "<Object_ID[]>"
  Bus Selector8/2 -> avoid_incomplete_trace2source13/1(In1)  "<Object_Type[]>"
  Bus Selector7/2 -> avoid_incomplete_trace2source11/1(In1)  "<Object_Type[]>"
  Bus Selector7/1 -> avoid_incomplete_trace2source10/1(In1)  "<Object_ID[]>"
  Bus Selector6/1 -> avoid_incomplete_trace2source8/1(In1)  "<Object_ID[]>"
  Bus Selector6/2 -> avoid_incomplete_trace2source9/1(In1)  "<Object_Type[]>"
  Bus Selector5/2 -> avoid_incomplete_trace2source7/1(In1)  "<Object_Type[]>"
  Bus Selector5/1 -> avoid_incomplete_trace2source6/1(In1)  "<Object_ID[]>"
  Sensor7/4(Object_Custom_Values[]) -> Terminator21/1
  Sensor7/2(Object_Position[]) -> Terminator19/1
  Sensor7/3(Object_Properties_Box[]) -> Terminator20/1
  Sensor6/3(Object_Properties_Box[]) -> Terminator17/1
  Sensor6/2(Object_Position[]) -> Terminator16/1
  Sensor6/4(Object_Custom_Values[]) -> Terminator18/1
  Sensor5/4(Object_Custom_Values[]) -> Terminator15/1
  Sensor5/2(Object_Position[]) -> Terminator13/1
  Sensor5/3(Object_Properties_Box[]) -> Terminator14/1
  Sensor4/3(Object_Properties_Box[]) -> Terminator11/1
  Sensor4/2(Object_Position[]) -> Terminator10/1
  Sensor4/4(Object_Custom_Values[]) -> Terminator12/1
  [ASMBUS_Environment_Traffic_Sensors_Object_Sensor_2D] -> Bus Selector4/1
  Sensor3/3(Object_Properties_Box[]) -> Terminator8/1
  Sensor3/2(Object_Position[]) -> Terminator7/1
  Sensor3/4(Object_Custom_Values[]) -> Terminator9/1
  Bus Selector3/1 -> avoid_incomplete_trace2source4/1(In1)  "<Object_ID[]>"
  Bus Selector3/2 -> avoid_incomplete_trace2source5/1(In1)  "<Object_Type[]>"
  Bus Selector4/3 -> Bus Selector3/1  "<Sensor_3_Left>"
  Bus Selector4/2 -> Bus Selector2/1  "<Sensor_2_Front_Left>"
  Bus Selector2/2 -> avoid_incomplete_trace2source3/1(In1)  "<Object_Type[]>"
  Bus Selector2/1 -> avoid_incomplete_trace2source2/1(In1)  "<Object_ID[]>"
  Sensor2/4(Object_Custom_Values[]) -> Terminator6/1
  Sensor2/2(Object_Position[]) -> Terminator1/1
  Sensor2/3(Object_Properties_Box[]) -> Terminator2/1
  Bus Selector4/1 -> Bus Selector1/1  "<Sensor_1_Front>"
  Road_Signals/1 -> Sensor1/4(Road_Signals), Sensor7/4(Road_Signals), Sensor6/4(Road_Signals), Sensor5/4(Road_Signals), Sensor4/4(Road_Signals), Sensor3/4(Road_Signals), Sensor2/4(Road_Signals)
  Traffic_Signals/1 -> Sensor1/3(Traffic_Signals), Sensor3/3(Traffic_Signals), Sensor4/3(Traffic_Signals), Sensor5/3(Traffic_Signals), Sensor6/3(Traffic_Signals), Sensor7/3(Traffic_Signals), Sensor2/3(Traffic_Signals)
  Bus Selector1/2 -> avoid_incomplete_trace2source1/1(In1)  "<Object_Type[]>"
  Sensor1/3(Object_Properties_Box[]) -> Terminator4/1
  Sensor1/2(Object_Position[]) -> Terminator3/1
  Bus Selector1/1 -> avoid_incomplete_trace2source/1(In1)  "<Object_ID[]>"
  Sensor1/4(Object_Custom_Values[]) -> Terminator5/1

== system ASM_Traffic/Environment/Sensors/PlantModel/Object_Sensor_2D/ScheduleAndCalculateSensor ==
  Enable_Init[0Off|1On] : Inport
  Sensor_Data[] : Inport  Port=2
  Enable[0Off|1On] : Inport  Port=3
  Traffic_Signals : Inport  Port=4
  Interface_In : Inport  Port=5
  Road_Signals : Inport  Port=6
  Bus Selector : BusSelector  OutputSignals=ExternalModel.Pos_Vehicle_CoorSys_E[x;y;z][m],ExternalModel.Angle_Vehicle_CoorSys_E[x;y;z][deg]
  Bus Selector1 : BusSelector  OutputSignals=Info.Flag_Sensor_Init_Ready[0|1]  OutputAsBus=on
  Bus Selector2 : BusSelector  OutputSignals=Plant.Traffic_Signals_toEnvironment.Flag_FellowUsed[0|1]
  Bus Selector3 : BusSelector  OutputSignals=Plant.ObjectParameters.FellowParameters.TrafficObject_Type_Fellows[],Plant.ObjectParameters.TrafficObjects.TrafficObject_Type_Data[],Plant.ObjectParameters.DiscreteObjects.DiscreteObject_Data[]
  Bus Selector4 : BusSelector  OutputSignals=Plant.TrafficObject_Data[]  OutputAsBus=on
  Bus Selector5 : BusSelector  OutputSignals=Plant.Traffic_Signals_toEnvironment
  Bus Selector6 : BusSelector  OutputSignals=Plant.ObjectParameters.TrafficObjects.TrafficObjectsState[],Plant.ObjectParameters.DiscreteObjects.DiscreteObjectsState[]
  GetFellowPositionVector : Subsystem
  Mux : Mux  Inputs=2
  Mux1 : Mux  Inputs=2
  OBJECT_SENSOR_2D_CALCULATION : ASM_Traffic_lib/Sensors/Object_Sensor_2D/OBJECT_SENSOR_2D_CALCULATION  Const_Sensor_Output_Dimension=MDL.Traffic.Sensors.ObjectSensor2D_Calculation.Const_Sensor_Output_Dimension  StepSize=SIM.StepSize  ASMProperties=struct('Name','OBJECT_SENSOR_2D_CALCULATION','Version','12.0','Library','ASM_Traffic_lib')  ASMInstanceName=object_sensor_2d_calculation  ASMInstanceID=1
  OBJECT_SENSOR_2D_PARAM_SELECTION : ASM_Traffic_lib/Sensors/Object_Sensor_2D/OBJECT_SENSOR_2D_PARAM_SELECTION  ASMProperties=struct('Name','OBJECT_SENSOR_2D_PARAM_SELECTION','Version','2.0','Library','ASM_Traffic_lib')  ASMInstanceName=object_sensor_2d_param_selection  ASMInstanceID=1
  OBJECT_SENSOR_2D_PARAM_VECTORIZATION : ASM_Traffic_lib/Sensors/Object_Sensor_2D/OBJECT_SENSOR_2D_PARAM_VECTORIZATION  ASMProperties=struct('Name','OBJECT_SENSOR_2D_PARAM_VECTORIZATION','Version','3.0','Library','ASM_Traffic_lib')  ASMInstanceName=object_sensor_2d_param_vectorization  ASMInstanceID=1
  SAMPLE_PULSE : ASM_Traffic_lib/Sensors/Scheduling/SAMPLE_PULSE  Tag=ASM_SUBCOMPONENT  Sw_SamplePulse=MDL.Traffic.Sensors.SamplePulse_2.Sw_SamplePulse  Const_t_Offs_Pulse=MDL.Traffic.Sensors.SamplePulse_2.Const_t_Offs_Pulse  Const_t_Cycle_Pulse=MDL.Traffic.Sensors.SamplePulse_2.Const_t_Cycle_Pulse  StepSize=SIM.StepSize  ASMProperties=struct('Name','SAMPLE_PULSE','Version','3.0','Library','ASM_Traffic_lib')  ASMInstanceName=sample_pulse  ASMInstanceID=2
      settings: AttributesFormatString=Instance Name: %<ASMInstanceName>\nInstance ID: %<ASMInstanceID>
  SENSOR_SCHEDULER : ASM_Traffic_lib/Sensors/Scheduling/SENSOR_SCHEDULER  StepSize=SIM.StepSize  ASMProperties=struct('Name','SENSOR_SCHEDULER','Version','4.0','Library','ASM_Traffic_lib')  ASMInstanceName=sensor_scheduler  ASMInstanceID=1
  SampleAndHold : Subsystem  TreatAsAtomicUnit=on
  Terminator{1..5} (5 alike) : Terminator
  SensorMapping_Data[] : Outport  VectorParamsAs1DForOutWhenUnconnected=off
  SensorSignals : Outport  Port=2  VectorParamsAs1DForOutWhenUnconnected=off
  Init_Ready[0Off|1On] : Outport  Port=3  VectorParamsAs1DForOutWhenUnconnected=off
  tag scope: ASMBUS_Environment_Traffic_SamplePulse_ObjectSensor2D=scoped, ASMBUS_Environment_Traffic_SensorScheduler_ObjectSensor2D=scoped
  wires:
  GetFellowPositionVector/1(Pos_Fellows_MainPnt_CoorSys_E[x;y;z][m]) -> SampleAndHold/3(In3)
  GetFellowPositionVector/2(Angle_Fellows[deg]) -> SampleAndHold/4(In4)
  Bus Selector5/1 -> GetFellowPositionVector/1(<FellowPositions>)  "<Traffic_Signals_toEnvironment>"
  OBJECT_SENSOR_2D_CALCULATION/2 -> Bus Selector1/1, SensorSignals/1
  Bus Selector1/1 -> Init_Ready[0Off|1On]/1
  Enable_Init[0Off|1On]/1 -> OBJECT_SENSOR_2D_CALCULATION/1
  SampleAndHold/2(Out2) -> OBJECT_SENSOR_2D_CALCULATION/6
  SampleAndHold/1(Out1) -> OBJECT_SENSOR_2D_CALCULATION/5
  SampleAndHold/4(Out4) -> OBJECT_SENSOR_2D_CALCULATION/8
  SampleAndHold/5(Out5) -> OBJECT_SENSOR_2D_CALCULATION/9
  SampleAndHold/3(Out3) -> OBJECT_SENSOR_2D_CALCULATION/7
  Bus Selector3/3 -> OBJECT_SENSOR_2D_CALCULATION/13  "<DiscreteObject_Data[]>"
  Mux/1 -> OBJECT_SENSOR_2D_CALCULATION/2
  SENSOR_SCHEDULER/9 -> Terminator4/1
  SENSOR_SCHEDULER/5 -> OBJECT_SENSOR_2D_CALCULATION/3
  Bus Selector2/1 -> SampleAndHold/5(In5)  "<Flag_FellowUsed[0|1]>"
  SENSOR_SCHEDULER/4 -> Mux/2
  SENSOR_SCHEDULER/3 -> Terminator5/1
  SENSOR_SCHEDULER/2 -> SensorMapping_Data[]/1
  SENSOR_SCHEDULER/6 -> OBJECT_SENSOR_2D_PARAM_SELECTION/1
  Traffic_Signals/1 -> Bus Selector5/1, Bus Selector2/1, Bus Selector3/1, Bus Selector6/1
  Interface_In/1 -> Bus Selector/1
  Bus Selector4/1 -> OBJECT_SENSOR_2D_CALCULATION/12
  Road_Signals/1 -> Bus Selector4/1
  Bus Selector3/2 -> OBJECT_SENSOR_2D_CALCULATION/11  "<TrafficObject_Type_Data[]>"
  Bus Selector/1 -> SampleAndHold/1(In1)  "<Pos_Vehicle_CoorSys_E[x;y;z][m]>"
  Bus Selector/2 -> SampleAndHold/2(In2)  "<Angle_Vehicle_CoorSys_E[x;y;z][deg]>"
  Bus Selector3/1 -> OBJECT_SENSOR_2D_CALCULATION/10  "<TrafficObject_Type_Fellows[]>"
  Sensor_Data[]/1 -> OBJECT_SENSOR_2D_PARAM_VECTORIZATION/1
  Enable[0Off|1On]/1 -> SAMPLE_PULSE/1, SENSOR_SCHEDULER/1, Mux/1
  SENSOR_SCHEDULER/7 -> Terminator2/1
  OBJECT_SENSOR_2D_CALCULATION/1 -> Terminator3/1
  OBJECT_SENSOR_2D_PARAM_SELECTION/1 -> OBJECT_SENSOR_2D_CALCULATION/4
  SENSOR_SCHEDULER/8 -> Terminator1/1
  SENSOR_SCHEDULER/1 -> [ASMBUS_Environment_Traffic_SensorScheduler_ObjectSensor2D]
  OBJECT_SENSOR_2D_PARAM_VECTORIZATION/1 -> SENSOR_SCHEDULER/2
  OBJECT_SENSOR_2D_PARAM_VECTORIZATION/2 -> OBJECT_SENSOR_2D_PARAM_SELECTION/2
  SAMPLE_PULSE/2 -> SampleAndHold/Enable
  SAMPLE_PULSE/1 -> [ASMBUS_Environment_Traffic_SamplePulse_ObjectSensor2D]
  Bus Selector6/2 -> Mux1/2  "<DiscreteObjectsState[]>"
  Bus Selector6/1 -> Mux1/1  "<TrafficObjectsState[]>"
  Mux1/1 -> OBJECT_SENSOR_2D_CALCULATION/14

== system ASM_Traffic/Environment/Sensors/PlantModel/Object_Sensor_2D/SensorMapping ==
  Enable[0Off|1On] : Inport
  SensorMapping_Data[] : Inport  Port=2
  SensorSignals : Inport  Port=3
  Bus Creator : BusCreator  Inputs=7
  Bus Selector : BusSelector  OutputSignals=Info
  Demux : Demux  Outputs=[4,4,4,4,4,4,4]
  OBJECT_SENSOR_2D_MAPPING{1..7} (7 alike) : ASM_Traffic_lib/Sensors/Object_Sensor_2D/OBJECT_SENSOR_2D_MAPPING  ASMProperties=struct('Name','OBJECT_SENSOR_2D_MAPPING','Version','1.0','Library','ASM_Traffic_lib')  ASMInstanceName=object_sensor_2d_mapping  ASMInstanceID=1
  Sensor_Signals : Outport  VectorParamsAs1DForOutWhenUnconnected=off
  tag scope: ASMBUS_Environment_Traffic_2DObjSensorCalc_Info=scoped, ASMBUS_Environment_Traffic_2DObjSensor_SensorSignals=scoped
  wires:
  Bus Creator/1 -> [ASMBUS_Environment_Traffic_2DObjSensor_SensorSignals]
  OBJECT_SENSOR_2D_MAPPING7/1 -> Bus Creator/7  "Sensor7"
  OBJECT_SENSOR_2D_MAPPING6/1 -> Bus Creator/6  "Sensor6"
  OBJECT_SENSOR_2D_MAPPING5/1 -> Bus Creator/5  "Sensor5"
  OBJECT_SENSOR_2D_MAPPING4/1 -> Bus Creator/4  "Sensor4"
  Demux/7 -> OBJECT_SENSOR_2D_MAPPING7/2
  Demux/6 -> OBJECT_SENSOR_2D_MAPPING6/2
  Demux/5 -> OBJECT_SENSOR_2D_MAPPING5/2
  Demux/4 -> OBJECT_SENSOR_2D_MAPPING4/2
  Enable[0Off|1On]/1 -> OBJECT_SENSOR_2D_MAPPING2/1, OBJECT_SENSOR_2D_MAPPING3/1, OBJECT_SENSOR_2D_MAPPING5/1, OBJECT_SENSOR_2D_MAPPING6/1, OBJECT_SENSOR_2D_MAPPING7/1, OBJECT_SENSOR_2D_MAPPING4/1, OBJECT_SENSOR_2D_MAPPING1/1
  SensorSignals/1 -> OBJECT_SENSOR_2D_MAPPING2/3, OBJECT_SENSOR_2D_MAPPING5/3, OBJECT_SENSOR_2D_MAPPING6/3, OBJECT_SENSOR_2D_MAPPING7/3, Bus Selector/1, OBJECT_SENSOR_2D_MAPPING4/3, OBJECT_SENSOR_2D_MAPPING3/3, OBJECT_SENSOR_2D_MAPPING1/3
  Bus Selector/1 -> [ASMBUS_Environment_Traffic_2DObjSensorCalc_Info]  "<Info>"
  Demux/2 -> OBJECT_SENSOR_2D_MAPPING2/2
  OBJECT_SENSOR_2D_MAPPING3/1 -> Bus Creator/3  "Sensor3"
  OBJECT_SENSOR_2D_MAPPING2/1 -> Bus Creator/2  "Sensor2"
  SensorMapping_Data[]/1 -> Demux/1
  OBJECT_SENSOR_2D_MAPPING1/1 -> Sensor_Signals/1, Bus Creator/1  "Sensor1"
  Demux/3 -> OBJECT_SENSOR_2D_MAPPING3/2
  Demux/1 -> OBJECT_SENSOR_2D_MAPPING1/2
